simulink model "evm4s_battery_test"  (R2025b)
settings: Solver=ode23t  StartTime=0.0  StopTime=20  MaxStep=0.002  RelTol=1e-3
InitFcn:
  | Ts = 0.01;   % EVM / AFE sample time [s], matches bmsTestPlatform FixedStep
  | Rload = 4.8;   % normal ~3.2 A load stays connected throughout
  | Vchg  = 19;    % strong enough to out-supply the load and still charge
  | Rchg  = 0.5;
undefined symbols (not defined in the file or in its folder): bat4s
libraries: fl_lib x4, nesl_utility x2, bat4s_lib x1, BQ76952EVM x1, bq76952Decode_lib x1, ee_lib x1
settings Model: Creator=SC-Br  LastModifiedBy=SC-Br

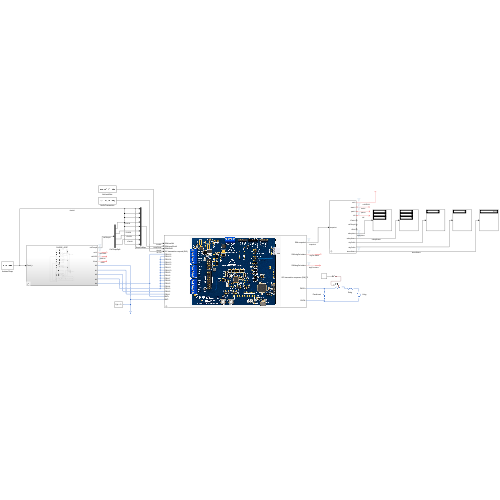
[thumbnail: Simulink's stored preview of the top-level diagram]
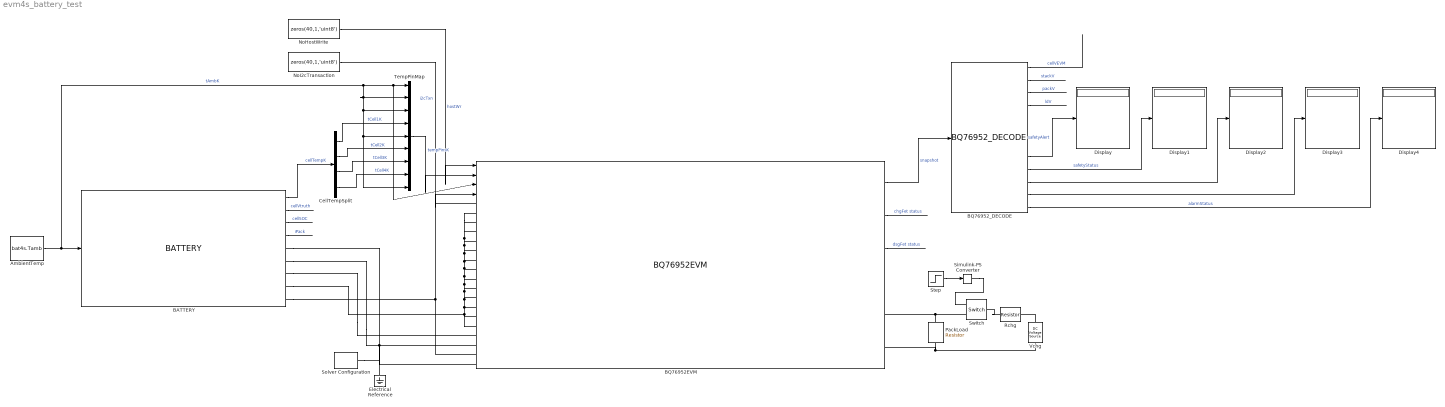
== system evm4s_battery_test ==
  AmbientTemp : Constant  Value=bat4s.Tamb
  BATTERY : bat4s_lib/BATTERY  SystemSampleTime=-1  VariantActivationTime=update diagram  EmptyChoice=off  PassThrough=off  PassThroughVariantControl=(default)  EmptyChoiceVariantControl=(default)  AllowFlexibleInterface=on  Latency=0  AutoFrameSizeCalculation=off
  BQ76952EVM : BQ76952EVM/BQ76952EVM  SeriesCount=4  UsedCellMask=32775  CellSenseOhms=20  CellFilterFarads=220e-9  PositiveLinkOhms=1e-6  Preset=Generic 4S  ShuntOhms=0.001  DAConfig=6  SampleTime=Ts  PinConfig=[0 0 0 7 0 7 7 7 0]  ProtEnabledA=188  ProtEnabledB=51  COV_Threshold=84  COV_Hyst=2  COV_Delay=74  CUV_Threshold=53  CUV_Hyst=2  CUV_Delay=74  OCC_Threshold=2  OCC_Delay=4  OCC_Recovery_mA=-200  OCD1_Threshold=5  OCD1_Delay=127  OCD_Recovery_mA=200  SCD_Threshold=1  SCD_Delay=2  SCD_Recovery_s=5  OTC_Threshold_C=45  OTC_Recovery_C=40  OTD_Threshold_C=60  OTD_Recovery_C=55  UTC_Threshold_C=0  UTC_Recovery_C=5  UTD_Threshold_C=-10  UTD_Recovery_C=-5  OTUT_Delay_s=2  RecoveryTime_s=3  MfgStatusInit=16  FetRon=0.001  FetGoff=1e-6  DisplayMode=PCB View  I2CAddress=8
  BQ76952_DECODE : bq76952Decode_lib/BQ76952_DECODE  DAConfig=6  cellMap=[1 2 3 16]  thermPins=[4 6 7 8]
  CellTempSplit : Demux
  Display{,1..4} (5 alike) : Display
  Electrical Reference : fl_lib/Electrical/Electrical Elements/Electrical Reference
  NoHostWrite : Constant  Value=zeros(40,1,'uint8')
  NoI2cTransaction : Constant  Value=zeros(40,1,'uint8')
  PackLoad : fl_lib/Electrical/Electrical Elements/Resistor  R=Rload Ohm  i_specify=off  i_priority=None  i=0 A  i_nominal_specify=off  i_nominal_value=1  i_nominal_unit=A  v_specify=off  v_priority=None  v=0 V  v_nominal_specify=off  v_nominal_value=1  v_nominal_unit=V
  Rchg : fl_lib/Electrical/Electrical Elements/Resistor  R=Rchg Ohm  i_specify=off  i_priority=None  i=0 A  i_nominal_specify=off  i_nominal_value=1  i_nominal_unit=A  v_specify=off  v_priority=None  v=0 V  v_nominal_specify=off  v_nominal_value=1  v_nominal_unit=V
  Simulink-PS Converter : nesl_utility/Simulink-PS Converter  PhysicalDomain=network_engine_domain  SubClassName=ps_input  LeftPortType=input  RightPortType=output  PseudoPeriodic=off  Frequencies=[]  NoiseDistribution=none  NoiseParameters=[]  Unit=1  AffineConversion=off  FilteringAndDerivatives=provide  SimscapeFilterOrder=1  InputFilterTimeConstant=0.001  UdotUserProvided=0
  Solver Configuration : nesl_utility/Solver Configuration  PhysicalDomain=network_engine_domain  SubClassName=solver  LeftPortType=input  RightPortType=generic  Tones=[]  Harmonics=[]  SimulateNoise=off  Profile=off  UseLocalSampling=off  EnableSwitchedLinearOptims=on  FrequencyDomain=off  UseCCode=off  RelTol=0.001  AbsTol=0.001  MinStep=1e-09  ToWorkspace=off  RevertToSquareIcSolve=off  NumHomotopyIterations=100  PhasorMode=off  PhasorModeNumHarmonics=1  ConsistencySolver=NEWTON_XTOL_AFTER_FTOL  IndexReductionMethod=DerivativeReplacement  DoDC=off  ResidualTolerance=1e-09  ConsistencyTolSource=GLOBAL  ConsistencyAbsTol=0.001  ConsistencyRelTol=0.001  ConsistencyTolFactor=0.001  UseLocalSolver=off  LocalSolverChoice=NE_BACKWARD_EULER_ADVANCER  ResolveIndetEquations=on  FunctionEvalNumThread=1  LocalSolverSampleTime=0.001  DoFixedCost=off  MaxNonlinIter=3  MaxModeIter=2  ComputeImpulses=off  ImpulseIterations=2  LinearAlgebra=auto  LinearAlgebraNumThread=0  EquationFormulation=NE_TIME_EF  DelaysMemoryBudget=1024  AutomaticFiltering=on  FilteringTimeConstant=0.001  PartitionStorageMethod=AS_NEEDED  PartitionMemoryBudget=1024  PartitionMethod=ROBUST  MultibodyUseLocalSolver=off  MultibodyLocalSolverChoice=ODE1  MultibodyLocalSolverSampleTime=0.001
  Step : Step  Time=5  Before=1  After=0  SampleTime=0
  Switch : fl_lib/Electrical/Electrical Elements/Switch  R_closed=0.01 Ohm  G_open=1e-8 1/Ohm  Threshold=0.5  i_specify=off  i_priority=None  i=0 A  i_nominal_specify=off  i_nominal_value=1  i_nominal_unit=A  v_specify=off  v_priority=None  v=0 V  v_nominal_specify=off  v_nominal_value=1  v_nominal_unit=V
  TempPinMap : Mux  Inputs=9
  Vchg : ee_lib/Additional Components/SPICE Sources/DC Voltage Source  DC=Vchg V
  wires:
  AmbientTemp/1 -> BQ76952EVM/3, TempPinMap/1, TempPinMap/3, TempPinMap/9, TempPinMap/5, TempPinMap/2, BATTERY/1  "tAmbK"
  BATTERY/1 -> CellTempSplit/1  "cellTempK"
  CellTempSplit/1 -> TempPinMap/4  "tCell1K"
  CellTempSplit/3 -> TempPinMap/7  "tCell3K"
  CellTempSplit/4 -> TempPinMap/8  "tCell4K"
  CellTempSplit/2 -> TempPinMap/6  "tCell2K"
  TempPinMap/1 -> BQ76952EVM/2  "tempPinsK"
  NoHostWrite/1 -> BQ76952EVM/1  "hostWr"
  NoI2cTransaction/1 -> BQ76952EVM/4  "i2cTxn"
  BATTERY/2 -> ?  "cellVtruth"
  BATTERY/3 -> ?  "cellSOC"
  BATTERY/4 -> ?  "iPack"
  BQ76952EVM/1 -> BQ76952_DECODE/1  "snapshot"
  BQ76952EVM/2 -> ?  "chgFet status"
  BQ76952EVM/3 -> ?  "dsgFet status"
  BQ76952_DECODE/8 -> Display/1  "safetyAlert"
  BQ76952_DECODE/9 -> Display1/1  "safetyStatus"
  BQ76952_DECODE/10 -> Display2/1
  BQ76952_DECODE/11 -> Display3/1
  BQ76952_DECODE/12 -> Display4/1  "alarmStatus"
  BQ76952_DECODE/2 -> ?  "stackV"
  BQ76952_DECODE/3 -> ?  "packV"
  BQ76952_DECODE/4 -> ?  "ldV"
  BQ76952_DECODE/1 -> ?  "cellVEVM"
  Step/1 -> Simulink-PS Converter/1
  connections:
  BATTERY/RConn1 -- Solver Configuration/RConn1 -- Electrical Reference/LConn1 -- BQ76952EVM/LConn18
  BATTERY/RConn2 -- BQ76952EVM/LConn16
  BATTERY/RConn3 -- BQ76952EVM/LConn15
  BATTERY/RConn4 -- BQ76952EVM/LConn3 -- BQ76952EVM/LConn2 -- BQ76952EVM/LConn4 -- BQ76952EVM/LConn5 -- BQ76952EVM/LConn6 -- BQ76952EVM/LConn7 -- BQ76952EVM/LConn8 -- BQ76952EVM/LConn9 -- BQ76952EVM/LConn10 -- BQ76952EVM/LConn11 -- BQ76952EVM/LConn12 -- BQ76952EVM/LConn13 -- BQ76952EVM/LConn14
  BATTERY/RConn5 -- BQ76952EVM/LConn17 -- BQ76952EVM/LConn1
  PackLoad/LConn1 -- BQ76952EVM/RConn1 -- Switch/RConn2
  PackLoad/RConn1 -- BQ76952EVM/RConn2 -- Vchg/RConn1
  Vchg/LConn1 -- Rchg/RConn1
  Rchg/LConn1 -- Switch/LConn1
  Simulink-PS Converter/RConn1 -- Switch/RConn1
